simulink model "lab3sim"  (R2025b)
settings: Solver=VariableStepAuto  StartTime=0.0  StopTime=50  MaxStep=1/1000  RelTol=1e-3
values from neighbouring files (symbols this model uses):
  A = [0, 1, 0, 0 ... (first row only)    [lab3.m]
  B = [0; 1/m1; 0; 0]    [lab3.m]
settings Model: Creator=dorian  LastModifiedBy=dorian

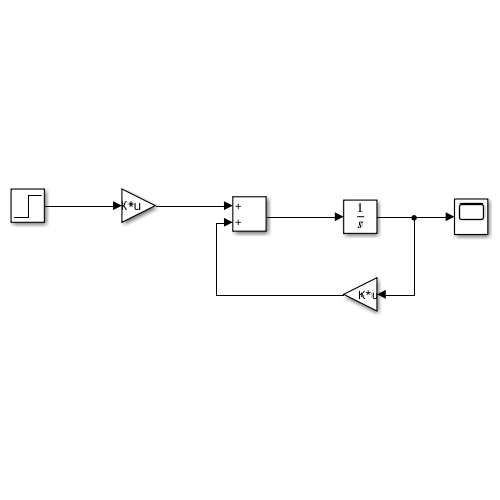
[thumbnail: Simulink's stored preview of the top-level diagram]
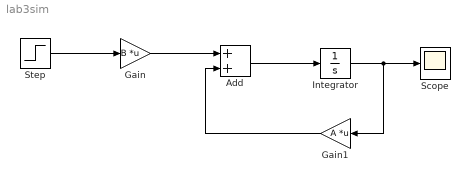
== system lab3sim ==
  Add : Sum
  Gain : Gain  Gain=B  Multiplication=Matrix(K*u)
  Gain1 : Gain  Gain=A  Multiplication=Matrix(K*u)
  Integrator : Integrator
  Scope : Scope
      settings: ActiveDisplayYMinimum=-52.247267466739885  ActiveDisplayYMaximum=140.79057677800091
  Step : Step  After=1000  SampleTime=0
  wires:
  Integrator/1 -> Gain1/1, Scope/1
  Add/1 -> Integrator/1
  Step/1 -> Gain/1
  Gain/1 -> Add/1
  Gain1/1 -> Add/2
